simulink model "SMXQ6_600_GoKart_Project"  (R2026a)
settings: Solver=VariableStepAuto  StopTime=7
model workspace (MAT data in the model file):
  CruiseSpeed = 1
  DaxisKi = 3000
  DaxisKp = 18
  InvThresh = 1
  MaxPower = 2638
  MaxTorque = 42
  NPP = 20
  QaxisKi = 3000
  QaxisKp = 18
  SpeedKi = 2882.18001217
  SpeedKp = 90.4773949421
  Tf = 0.0001
  Ts = 0.0001
  Vdc = 320
  flux = 0.103309826163
  speedramp = [0 0.125 0.125 0.5 0.5 1 1]
  timeramp = [0 1 2 3 4 5 6]
libraries: fl_lib x15, nesl_utility x15, sdl_lib x6, ee_lib x4, slpidlib x1, eePmsmFieldOrientedControl x1
(part 2 of 2)

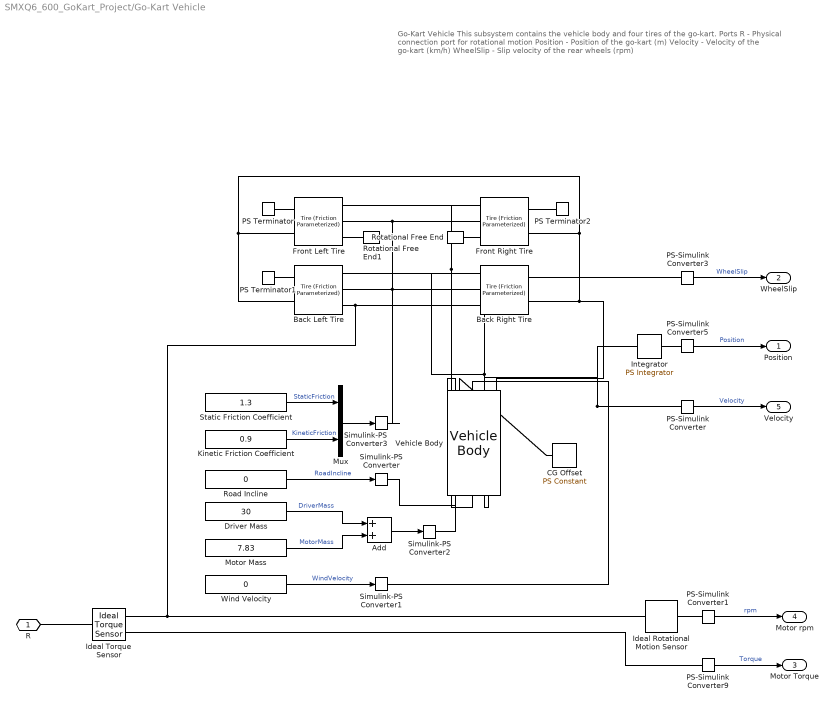
== system SMXQ6_600_GoKart_Project/Go-Kart Vehicle ==
  note: Go-Kart Vehicle
      |
      | This subsystem contains the vehicle body and four tires of the go-kart.
      |
      | Ports
      | R - Physical connection port for rotational motion
      | Position - Position of the go-kart (m)
      | Velocity - Velocity of the go-kart (km/h)
      | WheelSlip - Slip velocity of the rear wheels (rpm)
  Add : Sum
  Back Left Tire : sdl_lib/Tires & Vehicles/Tire (Friction Parameterized)  r_tire=0.25 m  slip_output=sdl.enum.SlipOutput.Absolute  friction_model=sdl.enum.friction_model_var.PS  mu_static=0.90  mu_kinetic=0.70  slip_vector=-flip([0, .02, .06, .15, .6, 1]) rad/s  mu_kinetic_vector=flip([.89, .88, .8, .75, .7, .7])  interp_method=simscape.enum.interpolation.linear  extrap_method=simscape.enum.extrapolation.linear  model_compliance=sdl.enum.compliance.off  stiffness=1e6 N/m  damping=1000 N*s/m  model_inertia=sdl.enum.model_inertia.off  wheel_inertia=0.7*(1) kg*m^2  belt_inertia=0.3*(1) kg*m^2  initial_velocity=0 rad/s  model_resistance=simscape.enum.onoff.off  resistance_model=sdl.enum.rollingResistanceParameterization.constant  coeff=0.015  p_tire=250e3 Pa  alpha=-0.003  beta=0.97  coeff_a=84e-4  coeff_b=6.2e-4 s/m  coeff_c=1.6e-4 s^2/m^2  v_thr=0.001 m/s  v_tol=0.01 m/s  F_min=10 N  initial_traction_state=sdl.enum.tireIC.traction
  Back Right Tire : sdl_lib/Tires & Vehicles/Tire (Friction Parameterized)  r_tire=0.25 m  slip_output=sdl.enum.SlipOutput.Absolute  friction_model=sdl.enum.friction_model_var.PS  mu_static=0.90  mu_kinetic=0.70  slip_vector=-flip([0, .02, .06, .15, .6, 1]) rad/s  mu_kinetic_vector=flip([.89, .88, .8, .75, .7, .7])  interp_method=simscape.enum.interpolation.linear  extrap_method=simscape.enum.extrapolation.linear  model_compliance=sdl.enum.compliance.off  stiffness=1e6 N/m  damping=1000 N*s/m  model_inertia=sdl.enum.model_inertia.off  wheel_inertia=0.7*(1) kg*m^2  belt_inertia=0.3*(1) kg*m^2  initial_velocity=0 rad/s  model_resistance=simscape.enum.onoff.off  resistance_model=sdl.enum.rollingResistanceParameterization.constant  coeff=0.015  p_tire=250e3 Pa  alpha=-0.003  beta=0.97  coeff_a=84e-4  coeff_b=6.2e-4 s/m  coeff_c=1.6e-4 s^2/m^2  v_thr=0.001 m/s  v_tol=0.01 m/s  F_min=10 N  initial_traction_state=sdl.enum.tireIC.traction
  CG Offset : fl_lib/Physical Signals/Sources/PS Constant  constant=0 m
  Driver Mass : Constant  Value=30
  Front Left Tire : sdl_lib/Tires & Vehicles/Tire (Friction Parameterized)  r_tire=0.25 m  slip_output=sdl.enum.SlipOutput.Absolute  friction_model=sdl.enum.friction_model_var.PS  mu_static=0.90  mu_kinetic=0.70  slip_vector=-flip([0, .02, .06, .15, .6, 1]) rad/s  mu_kinetic_vector=flip([.89, .88, .8, .75, .7, .7])  interp_method=simscape.enum.interpolation.linear  extrap_method=simscape.enum.extrapolation.linear  model_compliance=sdl.enum.compliance.off  stiffness=1e6 N/m  damping=1000 N*s/m  model_inertia=sdl.enum.model_inertia.off  wheel_inertia=0.7*(1) kg*m^2  belt_inertia=0.3*(1) kg*m^2  initial_velocity=0 rad/s  model_resistance=simscape.enum.onoff.off  resistance_model=sdl.enum.rollingResistanceParameterization.constant  coeff=0.015  p_tire=250e3 Pa  alpha=-0.003  beta=0.97  coeff_a=84e-4  coeff_b=6.2e-4 s/m  coeff_c=1.6e-4 s^2/m^2  v_thr=0.001 m/s  v_tol=0.01 m/s  F_min=10 N  initial_traction_state=sdl.enum.tireIC.traction
  Front Right Tire : sdl_lib/Tires & Vehicles/Tire (Friction Parameterized)  r_tire=0.25 m  slip_output=sdl.enum.SlipOutput.Absolute  friction_model=sdl.enum.friction_model_var.PS  mu_static=0.90  mu_kinetic=0.70  slip_vector=-flip([0, .02, .06, .15, .6, 1]) rad/s  mu_kinetic_vector=flip([.89, .88, .8, .75, .7, .7])  interp_method=simscape.enum.interpolation.linear  extrap_method=simscape.enum.extrapolation.linear  model_compliance=sdl.enum.compliance.off  stiffness=1e6 N/m  damping=1000 N*s/m  model_inertia=sdl.enum.model_inertia.off  wheel_inertia=0.7*(1) kg*m^2  belt_inertia=0.3*(1) kg*m^2  initial_velocity=0 rad/s  model_resistance=simscape.enum.onoff.off  resistance_model=sdl.enum.rollingResistanceParameterization.constant  coeff=0.015  p_tire=250e3 Pa  alpha=-0.003  beta=0.97  coeff_a=84e-4  coeff_b=6.2e-4 s/m  coeff_c=1.6e-4 s^2/m^2  v_thr=0.001 m/s  v_tol=0.01 m/s  F_min=10 N  initial_traction_state=sdl.enum.tireIC.traction
  Ideal Rotational Motion Sensor : fl_lib/Mechanical/Mechanical Sensors/Ideal Rotational Motion Sensor  reference=foundation.enum.MeasurementReference.absolute  acceleration_port=false  velocity_port=true  position_port=false  wrap_angle=false  offset=0 rad
  Ideal Torque Sensor : fl_lib/Mechanical/Mechanical Sensors/Ideal Torque Sensor
  Integrator : fl_lib/Physical Signals/Linear Operators/PS Integrator  reset_method=foundation.enum.IntegratorResetSpec.None  initial_condition_spec=foundation.enum.IntegratorICSpec.Internal  saturation_spec=foundation.enum.IntegratorSaturationSpec.None  saturation_source_spec=foundation.enum.IntegratorSaturationSourceSpec.Internal  x0=0 m  xu=inf s  xl=-inf s
  Kinetic Friction Coefficient : Constant  Value=0.9
  Motor Mass : Constant  Value=7.83
  Mux : Mux  Inputs=2
  PS Terminator : fl_lib/Physical Signals/Sinks/PS Terminator
  PS Terminator1 : fl_lib/Physical Signals/Sinks/PS Terminator
  PS Terminator2 : fl_lib/Physical Signals/Sinks/PS Terminator
  PS-Simulink Converter : nesl_utility/PS-Simulink Converter  PhysicalDomain=network_engine_domain  SubClassName=ps_output  LeftPortType=input  RightPortType=output  PseudoPeriodic=off  Frequencies=[]  VectorFormat=inherit  Unit=km/hr  AffineConversion=off
  PS-Simulink Converter1 : nesl_utility/PS-Simulink Converter  PhysicalDomain=network_engine_domain  SubClassName=ps_output  LeftPortType=input  RightPortType=output  PseudoPeriodic=off  Frequencies=[]  VectorFormat=inherit  Unit=rpm  AffineConversion=off
  PS-Simulink Converter3 : nesl_utility/PS-Simulink Converter  PhysicalDomain=network_engine_domain  SubClassName=ps_output  LeftPortType=input  RightPortType=output  PseudoPeriodic=off  Frequencies=[]  VectorFormat=inherit  Unit=rpm  AffineConversion=off
  PS-Simulink Converter5 : nesl_utility/PS-Simulink Converter  PhysicalDomain=network_engine_domain  SubClassName=ps_output  LeftPortType=input  RightPortType=output  PseudoPeriodic=off  Frequencies=[]  VectorFormat=inherit  Unit=m  AffineConversion=off
  PS-Simulink Converter9 : nesl_utility/PS-Simulink Converter  PhysicalDomain=network_engine_domain  SubClassName=ps_output  LeftPortType=input  RightPortType=output  PseudoPeriodic=off  Frequencies=[]  VectorFormat=inherit  Unit=inherit  AffineConversion=off
  Road Incline : Constant  Value=0
  Rotational Free End : fl_lib/Mechanical/Rotational Elements/Rotational Free End  w_specify=off  w_priority=None  w=0 rad/s  w_nominal_specify=off  w_nominal_value=1  w_nominal_unit=rad/s
  Rotational Free End1 : fl_lib/Mechanical/Rotational Elements/Rotational Free End  w_specify=off  w_priority=None  w=0 rad/s  w_nominal_specify=off  w_nominal_value=1  w_nominal_unit=rad/s
  Simulink-PS Converter : nesl_utility/Simulink-PS Converter  PhysicalDomain=network_engine_domain  SubClassName=ps_input  LeftPortType=input  RightPortType=output  PseudoPeriodic=off  Frequencies=[]  NoiseDistribution=none  NoiseParameters=[]  Unit=deg  AffineConversion=off  FilteringAndDerivatives=provide  SimscapeFilterOrder=1  InputFilterTimeConstant=0.001  UdotUserProvided=0
  Simulink-PS Converter1 : nesl_utility/Simulink-PS Converter  PhysicalDomain=network_engine_domain  SubClassName=ps_input  LeftPortType=input  RightPortType=output  PseudoPeriodic=off  Frequencies=[]  NoiseDistribution=none  NoiseParameters=[]  Unit=m/s  AffineConversion=off  FilteringAndDerivatives=provide  SimscapeFilterOrder=1  InputFilterTimeConstant=0.001  UdotUserProvided=0
  Simulink-PS Converter2 : nesl_utility/Simulink-PS Converter  PhysicalDomain=network_engine_domain  SubClassName=ps_input  LeftPortType=input  RightPortType=output  PseudoPeriodic=off  Frequencies=[]  NoiseDistribution=none  NoiseParameters=[]  Unit=kg  AffineConversion=off  FilteringAndDerivatives=provide  SimscapeFilterOrder=1  InputFilterTimeConstant=0.001  UdotUserProvided=0
  Simulink-PS Converter3 : nesl_utility/Simulink-PS Converter  PhysicalDomain=network_engine_domain  SubClassName=ps_input  LeftPortType=input  RightPortType=output  PseudoPeriodic=off  Frequencies=[]  NoiseDistribution=none  NoiseParameters=[]  Unit=1  AffineConversion=off  FilteringAndDerivatives=provide  SimscapeFilterOrder=1  InputFilterTimeConstant=0.001  UdotUserProvided=0
  Static Friction Coefficient : Constant  Value=1.3
  Vehicle Body : sdl_lib/Tires & Vehicles/Vehicle Body  mass=50 kg  n_w=2  x_f=0.9 m  x_r=0.3 m  y_c=0.1 m  mass_var=simscape.enum.onoff.on  g=9.81 m/s^2  liftoff_warning=simscape.enum.onoff.off  area=0.8 m^2  Cd_var=false  Cd=0.7  rho=1.1 kg/m^3  model_pitch=simscape.enum.onoff.off  inertia=4000 kg*m^2  suspension_model=sdl.enum.linearTLU.linear  k_f=1e4 N/m  b_f=1e4 N*s/m  k_r=1e4 N/m  b_r=1e4 N*s/m  k_f_TLU=[-2000, -1000, 0, 1000, 2000] N  x_f_TLU=[-.4, -.2, 0, .2, .4] m  b_f_TLU=[-200, -100, 0, 100, 200] N  v_f_TLU=[-4, -2, 0, 2, 4] m/s  k_r_TLU=[-2000, -1000, 0, 1000, 2000] N  x_r_TLU=[-.4, -.2, 0, .2, .4] m  b_r_TLU=[-200, -100, 0, 100, 200] N  v_r_TLU=[-4, -2, 0, 2, 4] m/s  interp_method=simscape.enum.interpolation.linear  extrap_method=simscape.enum.extrapolation.linear  model_hardstop=simscape.enum.onoff.off  upper_bound_f=.25 m  lower_bound_f=-.25 m  stop_k_f=1e6 N/m  stop_b_f=150 N*s/m  upper_bound_r=.25 m  lower_bound_r=-.25 m  stop_k_r=1e6 N/m  stop_b_r=150 N*s/m  initial_pitch=0 rad  initial_pitch_rate=0 rad/s  v_specify=off  v_priority=High  v=0 m/s  v_nominal_specify=off  v_nominal_value=1  v_nominal_unit=m/s
  Wind Velocity : Constant  Value=0
  R : PMIOPort  Side=Left
  Position : Outport  Unit=m
  WheelSlip : Outport  Port=2  Unit=rpm
  Motor Torque : Outport  Port=3  Unit=N*m
  Motor rpm : Outport  Port=4  Unit=rpm
  Velocity : Outport  Port=5  Unit=km/hr
  wires:
  Road Incline/1 -> Simulink-PS Converter/1  "RoadIncline"
  Wind Velocity/1 -> Simulink-PS Converter1/1  "WindVelocity"
  PS-Simulink Converter5/1 -> Position/1  "Position"
  PS-Simulink Converter3/1 -> WheelSlip/1  "WheelSlip"
  Static Friction Coefficient/1 -> Mux/1  "StaticFriction"
  Kinetic Friction Coefficient/1 -> Mux/2  "KineticFriction"
  Mux/1 -> Simulink-PS Converter3/1
  PS-Simulink Converter/1 -> Velocity/1  "Velocity"
  PS-Simulink Converter9/1 -> Motor Torque/1  "Torque"
  PS-Simulink Converter1/1 -> Motor rpm/1  "rpm"
  Driver Mass/1 -> Add/1  "DriverMass"
  Motor Mass/1 -> Add/2  "MotorMass"
  Add/1 -> Simulink-PS Converter2/1
  connections:
  Simulink-PS Converter1/RConn1 -- Vehicle Body/LConn3
  Vehicle Body/LConn5 -- Simulink-PS Converter2/RConn1
  PS-Simulink Converter/LConn1 -- Integrator/LConn1 -- Vehicle Body/LConn2
  Simulink-PS Converter/RConn1 -- Vehicle Body/RConn3
  Vehicle Body/LConn4 -- CG Offset/RConn1
  Vehicle Body/RConn2 -- Front Left Tire/LConn1 -- Front Right Tire/LConn1
  Vehicle Body/RConn1 -- Back Left Tire/LConn1 -- Back Right Tire/LConn1
  R/RConn1 -- Ideal Torque Sensor/LConn1
  Front Left Tire/RConn2 -- Back Left Tire/RConn2 -- Vehicle Body/LConn1 -- Back Right Tire/RConn2 -- Front Right Tire/RConn2
  Back Left Tire/RConn1 -- PS Terminator1/LConn1
  PS-Simulink Converter3/LConn1 -- Back Right Tire/RConn1
  PS Terminator2/LConn1 -- Front Right Tire/RConn1
  Rotational Free End/LConn1 -- Front Right Tire/LConn3
  Rotational Free End1/LConn1 -- Front Left Tire/LConn3
  Simulink-PS Converter3/RConn1 -- Front Left Tire/LConn2 -- Front Right Tire/LConn2 -- Back Left Tire/LConn2 -- Back Right Tire/LConn2
  PS-Simulink Converter5/LConn1 -- Integrator/RConn1
  PS Terminator/LConn1 -- Front Left Tire/RConn1
  PS-Simulink Converter9/LConn1 -- Ideal Torque Sensor/RConn2
  Back Left Tire/LConn3 -- Ideal Torque Sensor/RConn1 -- Ideal Rotational Motion Sensor/LConn1 -- Back Right Tire/LConn3
  PS-Simulink Converter1/LConn1 -- Ideal Rotational Motion Sensor/RConn1
